simulink model "fluids_chamber"  (R2026b)
settings: Solver=VariableStepAuto  StopTime=60*100
libraries: fl_lib x93, nesl_utility x21, ee_lib x12
(part 2 of 2)

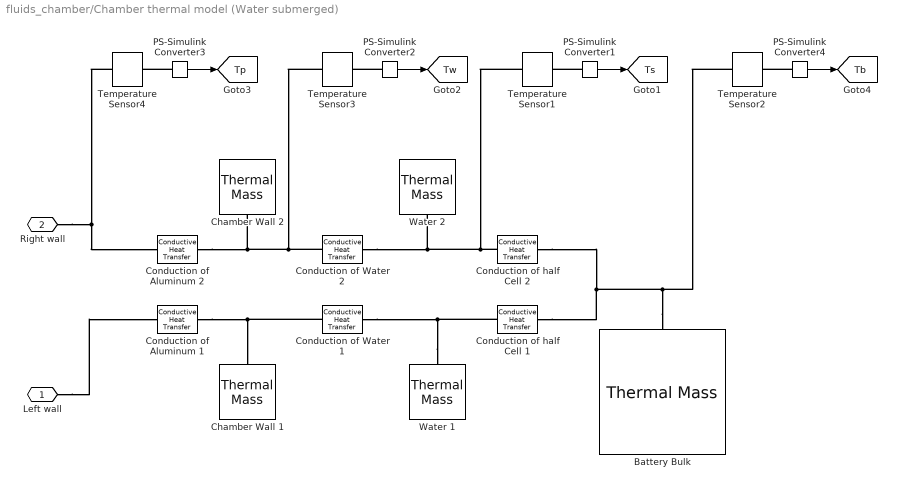
== system fluids_chamber/Chamber thermal model (Water submerged) ==
  Battery Bulk : fl_lib/Thermal/Thermal Elements/Thermal Mass  mass_type=foundation.enum.constant_variable.constant  mass=0.68 kg  sp_heat=1023 J/(K*kg)  mass_min=1e-6 kg  num_ports=foundation.enum.numPorts2.one  m_specify=off  m_priority=High  m=1 kg  m_nominal_specify=off  m_nominal_value=1  m_nominal_unit=kg  T_specify=on  T_priority=High  T=30+273 K  T_nominal_specify=off  T_nominal_value=1  T_nominal_unit=K  Q_specify=off  Q_priority=None  Q=0 W  Q_nominal_specify=off  Q_nominal_value=1  Q_nominal_unit=W
  Chamber Wall 1 : fl_lib/Thermal/Thermal Elements/Thermal Mass  mass_type=foundation.enum.constant_variable.constant  mass=0.1 kg  sp_heat=900 J/(K*kg)  mass_min=1e-6 kg  num_ports=foundation.enum.numPorts2.one  m_specify=off  m_priority=High  m=1 kg  m_nominal_specify=off  m_nominal_value=1  m_nominal_unit=kg  T_specify=on  T_priority=High  T=30+273 K  T_nominal_specify=off  T_nominal_value=1  T_nominal_unit=K  Q_specify=off  Q_priority=None  Q=0 W  Q_nominal_specify=off  Q_nominal_value=1  Q_nominal_unit=W
  Chamber Wall 2 : fl_lib/Thermal/Thermal Elements/Thermal Mass  mass_type=foundation.enum.constant_variable.constant  mass=0.1 kg  sp_heat=900 J/(K*kg)  mass_min=1e-6 kg  num_ports=foundation.enum.numPorts2.one  m_specify=off  m_priority=High  m=1 kg  m_nominal_specify=off  m_nominal_value=1  m_nominal_unit=kg  T_specify=on  T_priority=High  T=30+273 K  T_nominal_specify=off  T_nominal_value=1  T_nominal_unit=K  Q_specify=off  Q_priority=None  Q=0 W  Q_nominal_specify=off  Q_nominal_value=1  Q_nominal_unit=W
  Conduction of Aluminum 1 : fl_lib/Thermal/Thermal Elements/Conductive Heat Transfer  thermal_type=foundation.enum.ConstantVariableTabulated.Constant  wall_geometry=foundation.enum.ConductionWallGeometry.Planar  area=210*100 mm^2  thickness=1 mm  d_in=0.05 m  d_out=0.1 m  L=1 m  th_cond_min=10 W/(K*m)  th_cond=205 W/(K*m)  th_cond_TLU=[413, 401, 392, 383, 371, 357, 342] W/(K*m)  temp_TLU=[200, 273, 400, 600, 800, 1000, 1200] K  T_specify=off  T_priority=None  T=0 K  T_nominal_specify=off  T_nominal_value=1  T_nominal_unit=K  Q_specify=off  Q_priority=None  Q=0 W  Q_nominal_specify=off  Q_nominal_value=1  Q_nominal_unit=W
  Conduction of Aluminum 2 : fl_lib/Thermal/Thermal Elements/Conductive Heat Transfer  thermal_type=foundation.enum.ConstantVariableTabulated.Constant  wall_geometry=foundation.enum.ConductionWallGeometry.Planar  area=210*100 mm^2  thickness=1 mm  d_in=0.05 m  d_out=0.1 m  L=1 m  th_cond_min=10 W/(K*m)  th_cond=205 W/(K*m)  th_cond_TLU=[413, 401, 392, 383, 371, 357, 342] W/(K*m)  temp_TLU=[200, 273, 400, 600, 800, 1000, 1200] K  T_specify=off  T_priority=None  T=0 K  T_nominal_specify=off  T_nominal_value=1  T_nominal_unit=K  Q_specify=off  Q_priority=None  Q=0 W  Q_nominal_specify=off  Q_nominal_value=1  Q_nominal_unit=W
  Conduction of Water 1 : fl_lib/Thermal/Thermal Elements/Conductive Heat Transfer  thermal_type=foundation.enum.ConstantVariableTabulated.Constant  wall_geometry=foundation.enum.ConductionWallGeometry.Planar  area=210*100 mm^2  thickness=11 mm  d_in=0.05 m  d_out=0.1 m  L=1 m  th_cond_min=10 W/(K*m)  th_cond=0.6 W/(K*m)  th_cond_TLU=[413, 401, 392, 383, 371, 357, 342] W/(K*m)  temp_TLU=[200, 273, 400, 600, 800, 1000, 1200] K  T_specify=off  T_priority=None  T=0 K  T_nominal_specify=off  T_nominal_value=1  T_nominal_unit=K  Q_specify=off  Q_priority=None  Q=0 W  Q_nominal_specify=off  Q_nominal_value=1  Q_nominal_unit=W
  Conduction of Water 2 : fl_lib/Thermal/Thermal Elements/Conductive Heat Transfer  thermal_type=foundation.enum.ConstantVariableTabulated.Constant  wall_geometry=foundation.enum.ConductionWallGeometry.Planar  area=210*100 mm^2  thickness=11 mm  d_in=0.05 m  d_out=0.1 m  L=1 m  th_cond_min=10 W/(K*m)  th_cond=0.6 W/(K*m)  th_cond_TLU=[413, 401, 392, 383, 371, 357, 342] W/(K*m)  temp_TLU=[200, 273, 400, 600, 800, 1000, 1200] K  T_specify=off  T_priority=None  T=0 K  T_nominal_specify=off  T_nominal_value=1  T_nominal_unit=K  Q_specify=off  Q_priority=None  Q=0 W  Q_nominal_specify=off  Q_nominal_value=1  Q_nominal_unit=W
  Conduction of half Cell 1 : fl_lib/Thermal/Thermal Elements/Conductive Heat Transfer  thermal_type=foundation.enum.ConstantVariableTabulated.Constant  wall_geometry=foundation.enum.ConductionWallGeometry.Planar  area=180*70 mm^2  thickness=27/2 mm  d_in=0.05 m  d_out=0.1 m  L=1 m  th_cond_min=10 W/(K*m)  th_cond=0.91 W/(K*m)  th_cond_TLU=[413, 401, 392, 383, 371, 357, 342] W/(K*m)  temp_TLU=[200, 273, 400, 600, 800, 1000, 1200] K  T_specify=off  T_priority=None  T=0 K  T_nominal_specify=off  T_nominal_value=1  T_nominal_unit=K  Q_specify=off  Q_priority=None  Q=0 W  Q_nominal_specify=off  Q_nominal_value=1  Q_nominal_unit=W
  Conduction of half Cell 2 : fl_lib/Thermal/Thermal Elements/Conductive Heat Transfer  thermal_type=foundation.enum.ConstantVariableTabulated.Constant  wall_geometry=foundation.enum.ConductionWallGeometry.Planar  area=180*70 mm^2  thickness=27/2 mm  d_in=0.05 m  d_out=0.1 m  L=1 m  th_cond_min=10 W/(K*m)  th_cond=0.91 W/(K*m)  th_cond_TLU=[413, 401, 392, 383, 371, 357, 342] W/(K*m)  temp_TLU=[200, 273, 400, 600, 800, 1000, 1200] K  T_specify=off  T_priority=None  T=0 K  T_nominal_specify=off  T_nominal_value=1  T_nominal_unit=K  Q_specify=off  Q_priority=None  Q=0 W  Q_nominal_specify=off  Q_nominal_value=1  Q_nominal_unit=W
  PS-Simulink Converter{1..4} (4 alike) : nesl_utility/PS-Simulink Converter  PhysicalDomain=network_engine_domain  SubClassName=ps_output  LeftPortType=input  RightPortType=output  PseudoPeriodic=off  Frequencies=[]  VectorFormat=inherit  Unit=inherit  AffineConversion=off
  Temperature Sensor{1..4} (4 alike) : fl_lib/Thermal/Thermal Sensors/Temperature Sensor  temperature_measure=foundation.enum.MeasurementReference.absolute
  Water 1 : fl_lib/Thermal/Thermal Elements/Thermal Mass  mass_type=foundation.enum.constant_variable.constant  mass=0.71/2 kg  sp_heat=4180 J/(K*kg)  mass_min=1e-6 kg  num_ports=foundation.enum.numPorts2.one  m_specify=off  m_priority=High  m=1 kg  m_nominal_specify=off  m_nominal_value=1  m_nominal_unit=kg  T_specify=on  T_priority=High  T=30+273 K  T_nominal_specify=off  T_nominal_value=1  T_nominal_unit=K  Q_specify=off  Q_priority=None  Q=0 W  Q_nominal_specify=off  Q_nominal_value=1  Q_nominal_unit=W
  Water 2 : fl_lib/Thermal/Thermal Elements/Thermal Mass  mass_type=foundation.enum.constant_variable.constant  mass=0.71/2 kg  sp_heat=4180 J/(K*kg)  mass_min=1e-6 kg  num_ports=foundation.enum.numPorts2.one  m_specify=off  m_priority=High  m=1 kg  m_nominal_specify=off  m_nominal_value=1  m_nominal_unit=kg  T_specify=on  T_priority=High  T=30+273 K  T_nominal_specify=off  T_nominal_value=1  T_nominal_unit=K  Q_specify=off  Q_priority=None  Q=0 W  Q_nominal_specify=off  Q_nominal_value=1  Q_nominal_unit=W
  Left wall : PMIOPort  Side=Left
  Right wall : PMIOPort  Port=2  Side=Left
  tag scope: Tb=global, Tp=global, Ts=global, Tw=global
  wires:
  PS-Simulink Converter4/1 -> [Tb]
  PS-Simulink Converter3/1 -> [Tp]
  PS-Simulink Converter2/1 -> [Tw]
  PS-Simulink Converter1/1 -> [Ts]
  connections:
  Water 1/LConn1 -- Conduction of half Cell 1/LConn1 -- Conduction of Water 1/RConn1
  Conduction of Water 2/LConn1 -- Temperature Sensor3/LConn1 -- Conduction of Aluminum 2/RConn1 -- Chamber Wall 2/LConn1
  PS-Simulink Converter4/LConn1 -- Temperature Sensor2/RConn1
  Water 2/LConn1 -- Temperature Sensor1/LConn1 -- Conduction of half Cell 2/LConn1 -- Conduction of Water 2/RConn1
  Conduction of Water 1/LConn1 -- Conduction of Aluminum 1/RConn1 -- Chamber Wall 1/LConn1
  Battery Bulk/LConn1 -- Temperature Sensor2/LConn1 -- Conduction of half Cell 2/RConn1 -- Conduction of half Cell 1/RConn1
  PS-Simulink Converter3/LConn1 -- Temperature Sensor4/RConn1
  PS-Simulink Converter2/LConn1 -- Temperature Sensor3/RConn1
  Temperature Sensor4/LConn1 -- Right wall/RConn1 -- Conduction of Aluminum 2/LConn1
  PS-Simulink Converter1/LConn1 -- Temperature Sensor1/RConn1
  Left wall/RConn1 -- Conduction of Aluminum 1/LConn1

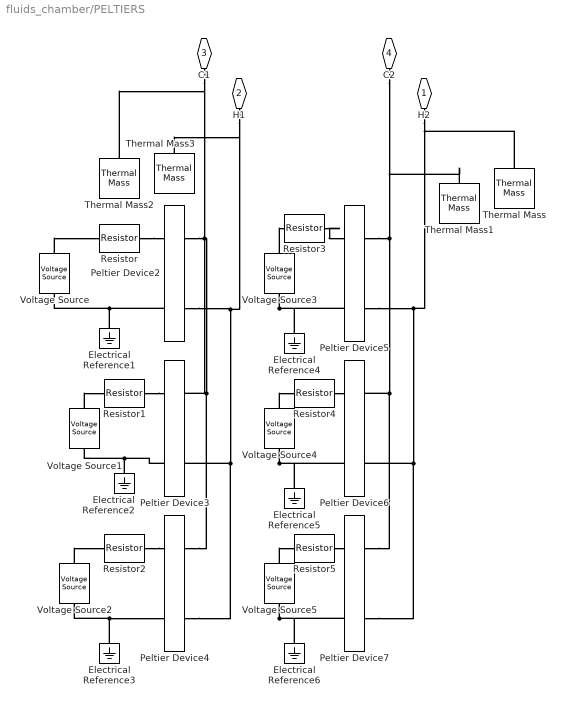
== system fluids_chamber/PELTIERS ==
  Electrical Reference{1..6} (6 alike) : fl_lib/Electrical/Electrical Elements/Electrical Reference
  Peltier Device{2..7} (6 alike) : ee_lib/Sensors & Transducers/Peltier Device  alpha=0.053 V/K  R=2 Ohm  K=1/2 W/K
  Resistor{,1..5} (6 alike) : fl_lib/Electrical/Electrical Elements/Resistor  R=rpel Ohm  i_specify=off  i_priority=None  i=0 A  i_nominal_specify=off  i_nominal_value=1  i_nominal_unit=A  v_specify=off  v_priority=None  v=0 V  v_nominal_specify=off  v_nominal_value=1  v_nominal_unit=V
  Thermal Mass{,1..3} (4 alike) : fl_lib/Thermal/Thermal Elements/Thermal Mass  mass_type=foundation.enum.constant_variable.constant  mass=(0.025/2)*3 kg  sp_heat=600 J/(K*kg)  mass_min=1e-6 kg  num_ports=foundation.enum.numPorts2.one  m_specify=off  m_priority=High  m=1 kg  m_nominal_specify=off  m_nominal_value=1  m_nominal_unit=kg  T_specify=on  T_priority=High  T=303 K  T_nominal_specify=off  T_nominal_value=1  T_nominal_unit=K  Q_specify=off  Q_priority=None  Q=0 W  Q_nominal_specify=off  Q_nominal_value=1  Q_nominal_unit=W
  Voltage Source : ee_lib/Sources/Voltage Source  dc_voltage=vpel V  ac_voltage=0 V  ac_shift=0 rad  ac_frequency=60 Hz  noise_mode=ee.enum.sources.noise.Disabled  PSD=0 V^2/Hz  sample_time=1e-3 s  repeatability=ee.enum.sources.repeatability.NotRepeatable  user_seed=0  auto_seed=3499211588  i_specify=off  i_priority=None  i=0 A  i_nominal_specify=off  i_nominal_value=1  i_nominal_unit=A  v_specify=off  v_priority=None  v=0 V  v_nominal_specify=off  v_nominal_value=1  v_nominal_unit=V
  Voltage Source1 : ee_lib/Sources/Voltage Source  dc_voltage=vpel V  ac_voltage=0 V  ac_shift=0 rad  ac_frequency=60 Hz  noise_mode=ee.enum.sources.noise.Disabled  PSD=0 V^2/Hz  sample_time=1e-3 s  repeatability=ee.enum.sources.repeatability.NotRepeatable  user_seed=0  auto_seed=3890346746  i_specify=off  i_priority=None  i=0 A  i_nominal_specify=off  i_nominal_value=1  i_nominal_unit=A  v_specify=off  v_priority=None  v=0 V  v_nominal_specify=off  v_nominal_value=1  v_nominal_unit=V
  Voltage Source2 : ee_lib/Sources/Voltage Source  dc_voltage=vpel V  ac_voltage=0 V  ac_shift=0 rad  ac_frequency=60 Hz  noise_mode=ee.enum.sources.noise.Disabled  PSD=0 V^2/Hz  sample_time=1e-3 s  repeatability=ee.enum.sources.repeatability.NotRepeatable  user_seed=0  auto_seed=545404223  i_specify=off  i_priority=None  i=0 A  i_nominal_specify=off  i_nominal_value=1  i_nominal_unit=A  v_specify=off  v_priority=None  v=0 V  v_nominal_specify=off  v_nominal_value=1  v_nominal_unit=V
  Voltage Source3 : ee_lib/Sources/Voltage Source  dc_voltage=vpel V  ac_voltage=0 V  ac_shift=0 rad  ac_frequency=60 Hz  noise_mode=ee.enum.sources.noise.Disabled  PSD=0 V^2/Hz  sample_time=1e-3 s  repeatability=ee.enum.sources.repeatability.NotRepeatable  user_seed=0  auto_seed=3922919431  i_specify=off  i_priority=None  i=0 A  i_nominal_specify=off  i_nominal_value=1  i_nominal_unit=A  v_specify=off  v_priority=None  v=0 V  v_nominal_specify=off  v_nominal_value=1  v_nominal_unit=V
  Voltage Source4 : ee_lib/Sources/Voltage Source  dc_voltage=vpel V  ac_voltage=0 V  ac_shift=0 rad  ac_frequency=60 Hz  noise_mode=ee.enum.sources.noise.Disabled  PSD=0 V^2/Hz  sample_time=1e-3 s  repeatability=ee.enum.sources.repeatability.NotRepeatable  user_seed=0  auto_seed=2715962282  i_specify=off  i_priority=None  i=0 A  i_nominal_specify=off  i_nominal_value=1  i_nominal_unit=A  v_specify=off  v_priority=None  v=0 V  v_nominal_specify=off  v_nominal_value=1  v_nominal_unit=V
  Voltage Source5 : ee_lib/Sources/Voltage Source  dc_voltage=vpel V  ac_voltage=0 V  ac_shift=0 rad  ac_frequency=60 Hz  noise_mode=ee.enum.sources.noise.Disabled  PSD=0 V^2/Hz  sample_time=1e-3 s  repeatability=ee.enum.sources.repeatability.NotRepeatable  user_seed=0  auto_seed=418932850  i_specify=off  i_priority=None  i=0 A  i_nominal_specify=off  i_nominal_value=1  i_nominal_unit=A  v_specify=off  v_priority=None  v=0 V  v_nominal_specify=off  v_nominal_value=1  v_nominal_unit=V
  H2 : PMIOPort  Side=Left
  H1 : PMIOPort  Port=2  Side=Left
  C1 : PMIOPort  Port=3  Side=Right
  C2 : PMIOPort  Port=4  Side=Right
  connections:
  Peltier Device7/RConn2 -- Peltier Device6/RConn2 -- Thermal Mass/LConn1 -- H2/RConn1 -- Peltier Device5/RConn2
  Peltier Device4/RConn1 -- Peltier Device3/RConn1 -- Thermal Mass2/LConn1 -- C1/RConn1 -- Peltier Device2/RConn1
  Peltier Device7/RConn1 -- Peltier Device6/RConn1 -- Thermal Mass1/LConn1 -- C2/RConn1 -- Peltier Device5/RConn1
  Peltier Device4/RConn2 -- Peltier Device3/RConn2 -- Thermal Mass3/LConn1 -- H1/RConn1 -- Peltier Device2/RConn2
  Electrical Reference1/LConn1 -- Voltage Source/RConn1 -- Peltier Device2/LConn2
  Electrical Reference2/LConn1 -- Peltier Device3/LConn2 -- Voltage Source1/RConn1
  Electrical Reference3/LConn1 -- Peltier Device4/LConn2 -- Voltage Source2/RConn1
  Voltage Source3/RConn1 -- Peltier Device5/LConn2 -- Electrical Reference4/LConn1
  Voltage Source4/RConn1 -- Peltier Device6/LConn2 -- Electrical Reference5/LConn1
  Voltage Source5/RConn1 -- Peltier Device7/LConn2 -- Electrical Reference6/LConn1
  Resistor/RConn1 -- Peltier Device2/LConn1
  Voltage Source/LConn1 -- Resistor/LConn1
  Resistor1/RConn1 -- Peltier Device3/LConn1
  Voltage Source1/LConn1 -- Resistor1/LConn1
  Resistor2/RConn1 -- Peltier Device4/LConn1
  Voltage Source2/LConn1 -- Resistor2/LConn1
  Voltage Source3/LConn1 -- Resistor3/LConn1
  Resistor3/RConn1 -- Peltier Device5/LConn1
  Voltage Source4/LConn1 -- Resistor4/LConn1
  Resistor4/RConn1 -- Peltier Device6/LConn1
  Resistor5/RConn1 -- Peltier Device7/LConn1
  Voltage Source5/LConn1 -- Resistor5/LConn1

== matlab function fluids_chamber/MATLAB Function ==
  data: u input; y output
function y = ktoc(u)

y = u-273;

== matlab function fluids_chamber/MATLAB Function2 ==
  data: u input; y output
function y = ktoc(u)

y = u-273;

== matlab function fluids_chamber/MATLAB Function3 ==
  data: u input; y output
function y = ktoc(u)

y = u-273;

== matlab function fluids_chamber/MATLAB Function4 ==
  data: u input; y output
function y = ktoc(u)

y = u-273;

== matlab function fluids_chamber/MATLAB Function5 ==
  data: u input; y output
function y = ktoc(u)

y = u-273;

== matlab function fluids_chamber/MATLAB Function1 ==
  data: u input; y output
function y = ktoc(u)

y = u-273;
